simulink model "drive_cmd_unpack"  (R2026b)
settings: Solver=VariableStepAuto
undefined symbols (not defined in the file or in its folder): P
libraries: simulink x5, svdutilitieslib x1
settings Model: Creator=aomar  LastModifiedBy=aomar

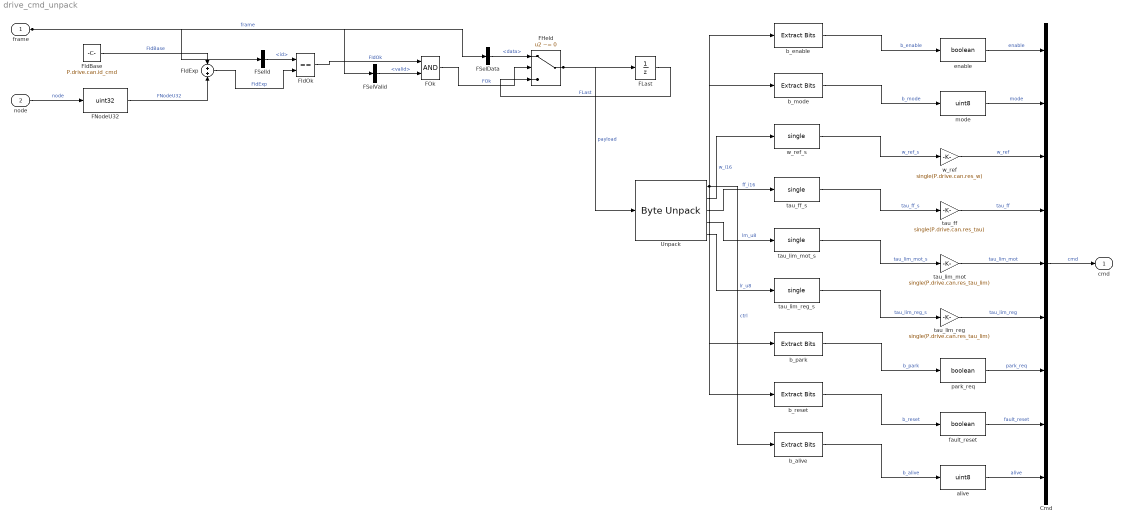
== system drive_cmd_unpack ==
  frame : Inport  OutDataTypeStr=Bus: Bus_CanFrame8
  node : Inport  Port=2  OutDataTypeStr=uint8
  Cmd : BusCreator  Inputs=9  OutDataTypeStr=Bus: Bus_DriveSideCmd  NonVirtualBus=on
  FHeld : Switch  Criteria=u2 ~= 0  SaturateOnIntegerOverflow=off  InputSameDT=off
  FIdBase : Constant  Value=P.drive.can.id_cmd  OutDataTypeStr=uint32
  FIdExp : Sum  OutDataTypeStr=uint32  SaturateOnIntegerOverflow=on
  FIdOk : RelationalOperator  Operator===  OutDataTypeStr=boolean  RndMeth=Simplest  InputSameDT=off
  FLast : UnitDelay  InitialCondition=zeros(8,1)  SampleTime=-1
  FNodeU32 : DataTypeConversion  OutDataTypeStr=uint32  RndMeth=Nearest
  FOk : Logic  AllPortsSameDT=off  OutDataTypeStr=boolean
  FSelData : BusSelector  OutputSignals=data
  FSelId : BusSelector  OutputSignals=id
  FSelValid : BusSelector  OutputSignals=valid
  Unpack : svdutilitieslib/Byte Unpack  dimensions={1,1,1,1,1}  datatypes={'uint16','int16','int16','uint8','uint8'}  byteAlign=1  blockPlatform=arduinoert
      settings: LibrarySourceBlock=mcblib/Signal Management/Byte Unpack
  alive : DataTypeConversion  OutDataTypeStr=uint8  RndMeth=Nearest
  b_alive : simulink/Logic and Bit Operations/Extract Bits  bitsToExtract=Range of bits  numBits=8  bitIdxRange=[8 15]  outScalingMode=Treat bit field as an integer
  b_enable : simulink/Logic and Bit Operations/Extract Bits  bitsToExtract=Range of bits  numBits=8  bitIdxRange=[0 0]  outScalingMode=Treat bit field as an integer
  b_mode : simulink/Logic and Bit Operations/Extract Bits  bitsToExtract=Range of bits  numBits=8  bitIdxRange=[3 4]  outScalingMode=Treat bit field as an integer
  b_park : simulink/Logic and Bit Operations/Extract Bits  bitsToExtract=Range of bits  numBits=8  bitIdxRange=[1 1]  outScalingMode=Treat bit field as an integer
  b_reset : simulink/Logic and Bit Operations/Extract Bits  bitsToExtract=Range of bits  numBits=8  bitIdxRange=[2 2]  outScalingMode=Treat bit field as an integer
  enable : DataTypeConversion  OutDataTypeStr=boolean  RndMeth=Nearest
  fault_reset : DataTypeConversion  OutDataTypeStr=boolean  RndMeth=Nearest
  mode : DataTypeConversion  OutDataTypeStr=uint8  RndMeth=Nearest
  park_req : DataTypeConversion  OutDataTypeStr=boolean  RndMeth=Nearest
  tau_ff : Gain  Gain=single(P.drive.can.res_tau)  ParamDataTypeStr=single  OutDataTypeStr=single
  tau_ff_s : DataTypeConversion  OutDataTypeStr=single  RndMeth=Nearest
  tau_lim_mot : Gain  Gain=single(P.drive.can.res_tau_lim)  ParamDataTypeStr=single  OutDataTypeStr=single
  tau_lim_mot_s : DataTypeConversion  OutDataTypeStr=single  RndMeth=Nearest
  tau_lim_reg : Gain  Gain=single(P.drive.can.res_tau_lim)  ParamDataTypeStr=single  OutDataTypeStr=single
  tau_lim_reg_s : DataTypeConversion  OutDataTypeStr=single  RndMeth=Nearest
  w_ref : Gain  Gain=single(P.drive.can.res_w)  ParamDataTypeStr=single  OutDataTypeStr=single
  w_ref_s : DataTypeConversion  OutDataTypeStr=single  RndMeth=Nearest
  cmd : Outport  OutDataTypeStr=Bus: Bus_DriveSideCmd
  wires:
  frame/1 -> FSelValid/1, FSelId/1, FSelData/1  "frame"
  node/1 -> FNodeU32/1  "node"
  FIdBase/1 -> FIdExp/1  "FIdBase"
  FNodeU32/1 -> FIdExp/2  "FNodeU32"
  FIdExp/1 -> FIdOk/2  "FIdExp"
  FSelId/1 -> FIdOk/1  "<id>"
  FIdOk/1 -> FOk/1  "FIdOk"
  FSelValid/1 -> FOk/2  "<valid>"
  FOk/1 -> FHeld/2  "FOk"
  FSelData/1 -> FHeld/1  "<data>"
  FHeld/1 -> Unpack/1, FLast/1  "payload"
  FLast/1 -> FHeld/3  "FLast"
  Unpack/1 -> b_alive/1, b_reset/1, b_park/1, b_enable/1, b_mode/1  "ctrl"
  Unpack/2 -> w_ref_s/1  "w_i16"
  Unpack/3 -> tau_ff_s/1  "ff_i16"
  Unpack/4 -> tau_lim_mot_s/1  "lm_u8"
  Unpack/5 -> tau_lim_reg_s/1  "lr_u8"
  w_ref_s/1 -> w_ref/1  "w_ref_s"
  tau_ff_s/1 -> tau_ff/1  "tau_ff_s"
  tau_lim_mot_s/1 -> tau_lim_mot/1  "tau_lim_mot_s"
  tau_lim_reg_s/1 -> tau_lim_reg/1  "tau_lim_reg_s"
  b_enable/1 -> enable/1  "b_enable"
  b_mode/1 -> mode/1  "b_mode"
  b_park/1 -> park_req/1  "b_park"
  b_reset/1 -> fault_reset/1  "b_reset"
  b_alive/1 -> alive/1  "b_alive"
  w_ref/1 -> Cmd/3  "w_ref"
  tau_ff/1 -> Cmd/4  "tau_ff"
  tau_lim_mot/1 -> Cmd/5  "tau_lim_mot"
  tau_lim_reg/1 -> Cmd/6  "tau_lim_reg"
  enable/1 -> Cmd/1  "enable"
  mode/1 -> Cmd/2  "mode"
  park_req/1 -> Cmd/7  "park_req"
  fault_reset/1 -> Cmd/8  "fault_reset"
  alive/1 -> Cmd/9  "alive"
  Cmd/1 -> cmd/1  "cmd"
